simulink model "snap_sys_clk_feng"  (R2019a)
settings: Solver=VariableStepDiscrete  StartTime=0.0  StopTime=10.0  RelTol=1e-3
undefined symbols (not defined in the file): datetime, posixtime
libraries: xbsIndex_r4 x5252, casper_library_misc x69, xps_library x6, casper_library_delays x3
(part 13 of 45)

== system snap_sys_clk_feng/stats/calc_adc_sum_sq7 ==
  note: 127^2 == 16129
  in : Inport
  Accumulator : xbsIndex_r4/Accumulator  operation=Add  n_bits=32  overflow=Wrap  scale=1  rst=on  hasbypass=on  infoeditControl=reset for floating point data type must be asserted for a minimum of 2 cycles  en=off  latency=1  msb_inp=100  msb=100  lsb=-100  use_behavioral_HDL=on  implementation=Fabric  dbl_ovrd=off  block_type=accum
      settings: xl_area=[0, 0, 0, 0, 0, 0, 0]  block_version=10.1.3
  Accumulator1 : xbsIndex_r4/Accumulator  operation=Add  n_bits=32  overflow=Wrap  scale=1  rst=on  hasbypass=on  infoeditControl=reset for floating point data type must be asserted for a minimum of 2 cycles  en=off  latency=1  msb_inp=100  msb=100  lsb=-100  use_behavioral_HDL=on  implementation=Fabric  dbl_ovrd=off  block_type=accum
      settings: xl_area=[0, 0, 0, 0, 0, 0, 0]  block_version=10.1.3
  Accumulator2 : xbsIndex_r4/Accumulator  operation=Add  n_bits=32  overflow=Wrap  scale=1  rst=on  hasbypass=on  infoeditControl=reset for floating point data type must be asserted for a minimum of 2 cycles  en=off  latency=1  msb_inp=100  msb=100  lsb=-100  use_behavioral_HDL=on  implementation=Fabric  dbl_ovrd=off  block_type=accum
      settings: xl_area=[0, 0, 0, 0, 0, 0, 0]  block_version=10.1.3
  BitBasher : xbsIndex_r4/BitBasher  bitexpr=sss={clip, s, ss}  display_expr=off  sr_1=sss  arith_type1="Signed  (2's comp)"  bin_pt1=0  sr_2=2  arith_type2=Unsigned  bin_pt2=0  sr_3=3  arith_type3=Unsigned  bin_pt3=0  sr_4=4  arith_type4=Unsigned  bin_pt4=0  dbl_ovrd=off  block_type=bitbasher
      settings: block_version=10.1.3
  Constant : xbsIndex_r4/Constant  const=127^2  gui_display_data_type=Fixed-point  arith_type=Unsigned  n_bits=15  bin_pt=0  preci_type=Single  exp_width=8  frac_width=24  explicit_period=on  period=1  equ=P=C  opselect=C  inp2=PCIN>>17  opr=+  inp1=P  carry=CIN  dbl_ovrd=off  block_type=constant
  Delay : xbsIndex_r4/Delay  rst=off  infoeditControl=Selection of Reset will increase slice count due to use of real FFs and instead of SRLs  en=off  latency=2  reg_retiming=off  dbl_ovrd=off  block_type=delay
  Delay1 : xbsIndex_r4/Delay  rst=off  infoeditControl=Selection of Reset will increase slice count due to use of real FFs and instead of SRLs  en=off  latency=1  reg_retiming=off  dbl_ovrd=off  block_type=delay
  Delay2 : xbsIndex_r4/Delay  rst=off  infoeditControl=Selection of Reset will increase slice count due to use of real FFs and instead of SRLs  en=off  latency=1  reg_retiming=off  dbl_ovrd=off  block_type=delay
      settings: infoedit=Hardware notes: A delay line is a chain, each link of which is an SRL16 or SRL32 followed by a flip-flop.
  Mult : xbsIndex_r4/Mult  precision=User Defined  arith_type=Unsigned  n_bits=15  bin_pt=0  quantization=Truncate  overflow=Wrap  en=off  latency=2  use_behavioral_HDL=on  opt=Speed  use_embedded=on  optimum_pipeline=on  pipeline=on  dbl_ovrd=off  use_rpm=on  placement_style=Rectangular shape  block_type=mult
      settings: xl_area=[0, 0, 0, 0, 0, 0, 0]  block_version=10.1.3
  Register : xbsIndex_r4/Register  init=0  rst=off  en=on  dbl_ovrd=off  block_type=register
      settings: xl_area=[0, 0, 0, 0, 0, 0, 0]
  Register1 : xbsIndex_r4/Register  init=0  rst=off  en=on  dbl_ovrd=off  block_type=register
      settings: xl_area=[0, 0, 0, 0, 0, 0, 0]
  Register2 : xbsIndex_r4/Register  init=0  rst=off  en=on  dbl_ovrd=off  block_type=register
      settings: xl_area=[0, 0, 0, 0, 0, 0, 0]
  Reinterpret : xbsIndex_r4/Reinterpret  force_arith_type=off  arith_type=Unsigned  force_bin_pt=on  bin_pt=0  block_type=reinterpret
  Relational : xbsIndex_r4/Relational  mode=a>=b  op_type=Ufix  en=off  latency=0  dbl_ovrd=off  block_type=relational
  sum_sumsq : Outport
  wires:
  Register2/1 -> BitBasher/1
  Register/1 -> BitBasher/3
  Register1/1 -> BitBasher/2
  Accumulator2/1 -> Register2/1
  Delay2/1 -> Register/2, Register1/2, Register2/2, Accumulator/2, Accumulator1/2, Accumulator2/2
  Relational/1 -> Accumulator2/1
  Constant/1 -> Relational/2
  Reinterpret/1 -> Delay1/1
  Delay1/1 -> Delay/1, Mult/1, Mult/2
  BitBasher/1 -> sum_sumsq/1
  Delay/1 -> Accumulator1/1
  Accumulator1/1 -> Register1/1
  Mult/1 -> Relational/1, Accumulator/1
  Accumulator/1 -> Register/1
  [adc_rms_rst] -> Delay2/1
  in/1 -> Reinterpret/1

== system snap_sys_clk_feng/stats/calc_adc_sum_sq8 ==
  note: 127^2 == 16129
  in : Inport
  Accumulator : xbsIndex_r4/Accumulator  operation=Add  n_bits=32  overflow=Wrap  scale=1  rst=on  hasbypass=on  infoeditControl=reset for floating point data type must be asserted for a minimum of 2 cycles  en=off  latency=1  msb_inp=100  msb=100  lsb=-100  use_behavioral_HDL=on  implementation=Fabric  dbl_ovrd=off  block_type=accum
      settings: xl_area=[0, 0, 0, 0, 0, 0, 0]  block_version=10.1.3
  Accumulator1 : xbsIndex_r4/Accumulator  operation=Add  n_bits=32  overflow=Wrap  scale=1  rst=on  hasbypass=on  infoeditControl=reset for floating point data type must be asserted for a minimum of 2 cycles  en=off  latency=1  msb_inp=100  msb=100  lsb=-100  use_behavioral_HDL=on  implementation=Fabric  dbl_ovrd=off  block_type=accum
      settings: xl_area=[0, 0, 0, 0, 0, 0, 0]  block_version=10.1.3
  Accumulator2 : xbsIndex_r4/Accumulator  operation=Add  n_bits=32  overflow=Wrap  scale=1  rst=on  hasbypass=on  infoeditControl=reset for floating point data type must be asserted for a minimum of 2 cycles  en=off  latency=1  msb_inp=100  msb=100  lsb=-100  use_behavioral_HDL=on  implementation=Fabric  dbl_ovrd=off  block_type=accum
      settings: xl_area=[0, 0, 0, 0, 0, 0, 0]  block_version=10.1.3
  BitBasher : xbsIndex_r4/BitBasher  bitexpr=sss={clip, s, ss}  display_expr=off  sr_1=sss  arith_type1="Signed  (2's comp)"  bin_pt1=0  sr_2=2  arith_type2=Unsigned  bin_pt2=0  sr_3=3  arith_type3=Unsigned  bin_pt3=0  sr_4=4  arith_type4=Unsigned  bin_pt4=0  dbl_ovrd=off  block_type=bitbasher
      settings: block_version=10.1.3
  Constant : xbsIndex_r4/Constant  const=127^2  gui_display_data_type=Fixed-point  arith_type=Unsigned  n_bits=15  bin_pt=0  preci_type=Single  exp_width=8  frac_width=24  explicit_period=on  period=1  equ=P=C  opselect=C  inp2=PCIN>>17  opr=+  inp1=P  carry=CIN  dbl_ovrd=off  block_type=constant
  Delay : xbsIndex_r4/Delay  rst=off  infoeditControl=Selection of Reset will increase slice count due to use of real FFs and instead of SRLs  en=off  latency=2  reg_retiming=off  dbl_ovrd=off  block_type=delay
  Delay1 : xbsIndex_r4/Delay  rst=off  infoeditControl=Selection of Reset will increase slice count due to use of real FFs and instead of SRLs  en=off  latency=1  reg_retiming=off  dbl_ovrd=off  block_type=delay
  Delay2 : xbsIndex_r4/Delay  rst=off  infoeditControl=Selection of Reset will increase slice count due to use of real FFs and instead of SRLs  en=off  latency=1  reg_retiming=off  dbl_ovrd=off  block_type=delay
      settings: infoedit=Hardware notes: A delay line is a chain, each link of which is an SRL16 or SRL32 followed by a flip-flop.
  Mult : xbsIndex_r4/Mult  precision=User Defined  arith_type=Unsigned  n_bits=15  bin_pt=0  quantization=Truncate  overflow=Wrap  en=off  latency=2  use_behavioral_HDL=on  opt=Speed  use_embedded=on  optimum_pipeline=on  pipeline=on  dbl_ovrd=off  use_rpm=on  placement_style=Rectangular shape  block_type=mult
      settings: xl_area=[0, 0, 0, 0, 0, 0, 0]  block_version=10.1.3
  Register : xbsIndex_r4/Register  init=0  rst=off  en=on  dbl_ovrd=off  block_type=register
      settings: xl_area=[0, 0, 0, 0, 0, 0, 0]
  Register1 : xbsIndex_r4/Register  init=0  rst=off  en=on  dbl_ovrd=off  block_type=register
      settings: xl_area=[0, 0, 0, 0, 0, 0, 0]
  Register2 : xbsIndex_r4/Register  init=0  rst=off  en=on  dbl_ovrd=off  block_type=register
      settings: xl_area=[0, 0, 0, 0, 0, 0, 0]
  Reinterpret : xbsIndex_r4/Reinterpret  force_arith_type=off  arith_type=Unsigned  force_bin_pt=on  bin_pt=0  block_type=reinterpret
  Relational : xbsIndex_r4/Relational  mode=a>=b  op_type=Ufix  en=off  latency=0  dbl_ovrd=off  block_type=relational
  sum_sumsq : Outport
  wires:
  Register2/1 -> BitBasher/1
  Register/1 -> BitBasher/3
  Register1/1 -> BitBasher/2
  Accumulator2/1 -> Register2/1
  Delay2/1 -> Register/2, Register1/2, Register2/2, Accumulator/2, Accumulator1/2, Accumulator2/2
  Relational/1 -> Accumulator2/1
  Constant/1 -> Relational/2
  Reinterpret/1 -> Delay1/1
  Delay1/1 -> Delay/1, Mult/1, Mult/2
  BitBasher/1 -> sum_sumsq/1
  Delay/1 -> Accumulator1/1
  Accumulator1/1 -> Register1/1
  Mult/1 -> Relational/1, Accumulator/1
  Accumulator/1 -> Register/1
  [adc_rms_rst] -> Delay2/1
  in/1 -> Reinterpret/1

== system snap_sys_clk_feng/stats/calc_adc_sum_sq9 ==
  note: 127^2 == 16129
  in : Inport
  Accumulator : xbsIndex_r4/Accumulator  operation=Add  n_bits=32  overflow=Wrap  scale=1  rst=on  hasbypass=on  infoeditControl=reset for floating point data type must be asserted for a minimum of 2 cycles  en=off  latency=1  msb_inp=100  msb=100  lsb=-100  use_behavioral_HDL=on  implementation=Fabric  dbl_ovrd=off  block_type=accum
      settings: xl_area=[0, 0, 0, 0, 0, 0, 0]  block_version=10.1.3
  Accumulator1 : xbsIndex_r4/Accumulator  operation=Add  n_bits=32  overflow=Wrap  scale=1  rst=on  hasbypass=on  infoeditControl=reset for floating point data type must be asserted for a minimum of 2 cycles  en=off  latency=1  msb_inp=100  msb=100  lsb=-100  use_behavioral_HDL=on  implementation=Fabric  dbl_ovrd=off  block_type=accum
      settings: xl_area=[0, 0, 0, 0, 0, 0, 0]  block_version=10.1.3
  Accumulator2 : xbsIndex_r4/Accumulator  operation=Add  n_bits=32  overflow=Wrap  scale=1  rst=on  hasbypass=on  infoeditControl=reset for floating point data type must be asserted for a minimum of 2 cycles  en=off  latency=1  msb_inp=100  msb=100  lsb=-100  use_behavioral_HDL=on  implementation=Fabric  dbl_ovrd=off  block_type=accum
      settings: xl_area=[0, 0, 0, 0, 0, 0, 0]  block_version=10.1.3
  BitBasher : xbsIndex_r4/BitBasher  bitexpr=sss={clip, s, ss}  display_expr=off  sr_1=sss  arith_type1="Signed  (2's comp)"  bin_pt1=0  sr_2=2  arith_type2=Unsigned  bin_pt2=0  sr_3=3  arith_type3=Unsigned  bin_pt3=0  sr_4=4  arith_type4=Unsigned  bin_pt4=0  dbl_ovrd=off  block_type=bitbasher
      settings: block_version=10.1.3
  Constant : xbsIndex_r4/Constant  const=127^2  gui_display_data_type=Fixed-point  arith_type=Unsigned  n_bits=15  bin_pt=0  preci_type=Single  exp_width=8  frac_width=24  explicit_period=on  period=1  equ=P=C  opselect=C  inp2=PCIN>>17  opr=+  inp1=P  carry=CIN  dbl_ovrd=off  block_type=constant
  Delay : xbsIndex_r4/Delay  rst=off  infoeditControl=Selection of Reset will increase slice count due to use of real FFs and instead of SRLs  en=off  latency=2  reg_retiming=off  dbl_ovrd=off  block_type=delay
  Delay1 : xbsIndex_r4/Delay  rst=off  infoeditControl=Selection of Reset will increase slice count due to use of real FFs and instead of SRLs  en=off  latency=1  reg_retiming=off  dbl_ovrd=off  block_type=delay
  Delay2 : xbsIndex_r4/Delay  rst=off  infoeditControl=Selection of Reset will increase slice count due to use of real FFs and instead of SRLs  en=off  latency=1  reg_retiming=off  dbl_ovrd=off  block_type=delay
      settings: infoedit=Hardware notes: A delay line is a chain, each link of which is an SRL16 or SRL32 followed by a flip-flop.
  Mult : xbsIndex_r4/Mult  precision=User Defined  arith_type=Unsigned  n_bits=15  bin_pt=0  quantization=Truncate  overflow=Wrap  en=off  latency=2  use_behavioral_HDL=on  opt=Speed  use_embedded=on  optimum_pipeline=on  pipeline=on  dbl_ovrd=off  use_rpm=on  placement_style=Rectangular shape  block_type=mult
      settings: xl_area=[0, 0, 0, 0, 0, 0, 0]  block_version=10.1.3
  Register : xbsIndex_r4/Register  init=0  rst=off  en=on  dbl_ovrd=off  block_type=register
      settings: xl_area=[0, 0, 0, 0, 0, 0, 0]
  Register1 : xbsIndex_r4/Register  init=0  rst=off  en=on  dbl_ovrd=off  block_type=register
      settings: xl_area=[0, 0, 0, 0, 0, 0, 0]
  Register2 : xbsIndex_r4/Register  init=0  rst=off  en=on  dbl_ovrd=off  block_type=register
      settings: xl_area=[0, 0, 0, 0, 0, 0, 0]
  Reinterpret : xbsIndex_r4/Reinterpret  force_arith_type=off  arith_type=Unsigned  force_bin_pt=on  bin_pt=0  block_type=reinterpret
  Relational : xbsIndex_r4/Relational  mode=a>=b  op_type=Ufix  en=off  latency=0  dbl_ovrd=off  block_type=relational
  sum_sumsq : Outport
  wires:
  in/1 -> Reinterpret/1
  [adc_rms_rst] -> Delay2/1
  Accumulator/1 -> Register/1
  Mult/1 -> Accumulator/1, Relational/1
  Accumulator1/1 -> Register1/1
  Delay/1 -> Accumulator1/1
  BitBasher/1 -> sum_sumsq/1
  Delay1/1 -> Mult/2, Mult/1, Delay/1
  Reinterpret/1 -> Delay1/1
  Constant/1 -> Relational/2
  Relational/1 -> Accumulator2/1
  Delay2/1 -> Accumulator2/2, Accumulator1/2, Accumulator/2, Register2/2, Register1/2, Register/2
  Accumulator2/1 -> Register2/1
  Register1/1 -> BitBasher/2
  Register/1 -> BitBasher/3
  Register2/1 -> BitBasher/1

== system snap_sys_clk_feng/stats/edge_detect ==
  in : Inport
  Delay : xbsIndex_r4/Delay  rst=off  infoeditControl=Selection of Reset will increase slice count due to use of real FFs and instead of SRLs  en=off  latency=1  reg_retiming=off  dbl_ovrd=off  block_type=delay
      settings: xl_area=[0, 0, 0, 0, 0, 0, 0]
  Inverter : xbsIndex_r4/Inverter  en=off  latency=0  dbl_ovrd=off  block_type=inv
      settings: xl_area=[0, 0, 0, 0, 0, 0, 0]
  edge_op : xbsIndex_r4/Logical  logical_function=NOR  inputs=2  en=off  latency=0  precision=Full  arith_type=Unsigned  n_bits=8  bin_pt=2  align_bp=on  dbl_ovrd=off  block_type=logical
      settings: xl_area=[0, 0, 0, 0, 0, 0, 0]
  out : Outport
  wires:
  Inverter/1 -> edge_op/1
  edge_op/1 -> out/1
  in/1 -> Inverter/1, Delay/1
  Delay/1 -> edge_op/2

== system snap_sys_clk_feng/stats/enable ==
  sim_1 : Inport
  convert1_1 : DataTypeConversion  OutDataTypeStr=fixdt('ufix32_En0')  LockScale=on
  convert2_1 : DataTypeConversion  OutDataTypeStr=fixdt('ufix32_En0')  ConvertRealWorld=Stored Integer (SI)  LockScale=on
  gain_1 : Gain
  io_delay : xbsIndex_r4/Delay  rst=off  infoeditControl=Selection of Reset will increase slice count due to use of real FFs and instead of SRLs  en=off  latency=0  reg_retiming=on  dbl_ovrd=off  block_type=delay
  reint1 : xbsIndex_r4/Reinterpret  force_arith_type=on  arith_type=Unsigned  force_bin_pt=on  bin_pt=0  block_type=reinterpret
  slice_reg : xbsIndex_r4/Slice  nbits=32  boolean_output=off  mode=Lower Bit Location + Width  bit1=0  base1=MSB of Input  bit0=0  base0=LSB of Input  dbl_ovrd=off  block_type=slice
  snap_sys_clk_feng_stats_enable_user_data_out : xbsIndex_r4/Gateway In  gui_display_data_type=Fixed-point  arith_type=Unsigned  n_bits=32  bin_pt=0  preci_type=Single  exp_width=8  frac_width=24  rows=1  columns=1  quantization="Round  (unbiased: +/- Inf)"  overflow=Saturate  period=1  UseAsADC=off  ADCChannel='1'  interface=None  automatic_assignment=on  address_offset=hex2dec('00')  intf_name=''  intf_description=''  default_value=0  timing_constraint=None  locs_specified=off  LOCs={}  io_standard={}  inherit_from_input=off  hdl_port=on  dbl_ovrd=off  block_type=gatewayin
  in_reg : Outport
  wires:
  snap_sys_clk_feng_stats_enable_user_data_out/1 -> io_delay/1
  sim_1/1 -> convert1_1/1
  convert1_1/1 -> convert2_1/1
  convert2_1/1 -> gain_1/1
  gain_1/1 -> snap_sys_clk_feng_stats_enable_user_data_out/1
  io_delay/1 -> slice_reg/1
  slice_reg/1 -> reint1/1
  reint1/1 -> in_reg/1

== system snap_sys_clk_feng/stats/levels ==
  addr : Inport
  data_in : Inport  Port=2
  we : Inport  Port=3
  Terminator : Terminator
  Terminator1 : Terminator
  Terminator2 : Terminator
  calc_add : Subsystem  mask{data_width=128, addr_width=5, sample_rate=sample_rate}
      mask prompts: data_width "data width"; addr_width "address width"; sample_rate "sample rate"
  convert_addr : xbsIndex_r4/Convert  gui_display_data_type=Fixed-point  arith_type=Unsigned  n_bits=addr_width  bin_pt=0  float_type=Single  exp_bits=8  fraction_bits=24  quantization=Truncate  overflow=Wrap  en=off  latency=0  pipeline=off  dbl_ovrd=off  block_type=convert
      settings: xl_area=[0, 0, 0, 0, 0, 0, 0]
  convert_din1 : xbsIndex_r4/Convert  gui_display_data_type=Fixed-point  arith_type=Unsigned  n_bits=128  bin_pt=0  float_type=Single  exp_bits=8  fraction_bits=24  quantization=Truncate  overflow=Wrap  en=off  latency=0  pipeline=off  dbl_ovrd=off  block_type=convert
      settings: xl_area=[0, 0, 0, 0, 0, 0, 0]
  convert_we : xbsIndex_r4/Convert  gui_display_data_type=Fixed-point  arith_type=Unsigned  n_bits=1  bin_pt=0  float_type=Single  exp_bits=8  fraction_bits=24  quantization=Truncate  overflow=Wrap  en=off  latency=0  pipeline=off  dbl_ovrd=off  block_type=convert
      settings: xl_area=[0, 0, 0, 0, 0, 0, 0]
  munge_in : Subsystem  AncestorBlock=casper_library_flow_control/munge  mask(munge){divisions=4, div_size=[32 32 32 32], order=[3  2  1  0], arith_type_out=Unsigned, bin_pt_out=0}
      mask prompts: divisions "Number of divisions"; div_size "Division size (bits)"; order "Division packing order"; arith_type_out "Output arithmetic type"; bin_pt_out "Output binary point"
      mask help: Splits an input bus into the specified number of divisions and then recombines them in the order specified (most significant division = 0,least = number divisions-1)
      mask init:
      | munge_init(gcb, ...
      |     'divisions', divisions, ...
      |     'div_size', div_size, ...
      |     'order', order, ...
      |     'arith_type_out', arith_type_out, ...
      |     'bin_pt_out', bin_pt_out);
      settings: AttributesFormatString=|
      | split:[32 32 32 32]
      | join:[3 2 1 0]
      | Unsigned [128,0]
      mask TypeOptions arith_type_out: Unsigned | Signed  (2's comp) | Floating-point
  munge_out : Subsystem  AncestorBlock=casper_library_flow_control/munge  mask(munge){divisions=4, div_size=[32 32 32 32], order=[3  2  1  0], arith_type_out=Unsigned, bin_pt_out=0}
      mask prompts: divisions "Number of divisions"; div_size "Division size (bits)"; order "Division packing order"; arith_type_out "Output arithmetic type"; bin_pt_out "Output binary point"
      mask help: Splits an input bus into the specified number of divisions and then recombines them in the order specified (most significant division = 0,least = number divisions-1)
      mask init:
      | munge_init(gcb, ...
      |     'divisions', divisions, ...
      |     'div_size', div_size, ...
      |     'order', order, ...
      |     'arith_type_out', arith_type_out, ...
      |     'bin_pt_out', bin_pt_out);
      settings: AttributesFormatString=|
      | split:[32 32 32 32]
      | join:[3 2 1 0]
      | Unsigned [128,0]
      mask TypeOptions arith_type_out: Unsigned | Signed  (2's comp) | Floating-point
  sim_mem : Subsystem  mask{arith_type=Unsigned, addr_width=5, data_width=128, data_bin_pt=0, init_vals=[0   1   2   3   4   5   6   7   8   9  10  11  12  13  14  15  16  17  18  19  20  21  22  23  24  25  26  27  28  29  30  31], sample_rate=1, csp_latency=3}
      mask prompts: arith_type "Output Data Type"; addr_width "Address width"; data_width "Data width"; data_bin_pt "Data Binary Point"; init_vals "Initial values"; sample_rate "Sample rate"; csp_latency "Latency"
      mask init:
      | % set_param([gcb, '/data_to_xilinx'], 'arith_type', arith_type)
      | % set_param([gcb, '/data_to_xilinx'], 'n_bits', get_param(gcb, 'data_width'))
      mask TypeOptions arith_type: Unsigned | Signed  (2's comp)
      mask TypeOptions data_width: 8 | 16 | 32 | 64 | 128
  snap_sys_clk_feng_stats_levels_addr : xbsIndex_r4/Gateway Out  inherit_from_input=off  hdl_port=on  rows=1  columns=1  UseAsDAC=off  DACChannel='1'  interface=None  automatic_assignment=on  address_offset=hex2dec('00')  intf_name=''  intf_description=''  timing_constraint=None  locs_specified=off  LOCs={'A5','B9','A9','C1','A3','G6','E9','A6','A7','A8','B8','B1','B3','D9','B5','B4','B6','C2'}  io_standard={}  block_type=gatewayout
      settings: infoedit="Gateway out block.  Converts Xilinx fixed point inputs into ouputs of type Simulink integer, double, or fixed point.<P><P>Hardware notes:  In hardware these blocks become top level output ports or are discarded, depending on how they are configured."  sginterface={'Nallatech'=>{'xdspkit'=>{'non_memory_mapped_port'=>'uprev_Shared_BRAM_addr'}},'Xilinx'=>{'jtaghwcosim'=>{'non_memory_mapped_port'=>'uprev_Shared_BRAM_addr'},'xdspkit'=>{'non_memory_mapped_port'=>'uprev_Shared_BRAM_addr'}}}  xl_area=[0, 0, 0, 0, 0, 0, 0]
  snap_sys_clk_feng_stats_levels_data_in : xbsIndex_r4/Gateway Out  inherit_from_input=off  hdl_port=on  rows=1  columns=1  UseAsDAC=off  DACChannel='1'  interface=None  automatic_assignment=on  address_offset=hex2dec('00')  intf_name=''  intf_description=''  timing_constraint=None  locs_specified=off  LOCs={'B21','B22','A22','B23','B19','C19','A20','A21','A23','B24','A24','A25','E18','D18','C18','B18'}  io_standard={}  block_type=gatewayout
      settings: infoedit="Gateway out block.  Converts Xilinx fixed point inputs into ouputs of type Simulink integer, double, or fixed point.<P><P>Hardware notes:  In hardware these blocks become top level output ports or are discarded, depending on how they are configured."  sginterface={'Nallatech'=>{'xdspkit'=>{'non_memory_mapped_port'=>'uprev_Shared_BRAM_data_in'}},'Xilinx'=>{'jtaghwcosim'=>{'non_memory_mapped_port'=>'uprev_Shared_BRAM_data_in'},'xdspkit'=>{'non_memory_mapped_port'=>'uprev_Shared_BRAM_data_in'}}}  xl_area=[0, 0, 0, 0, 0, 0, 0]
  snap_sys_clk_feng_stats_levels_data_out : xbsIndex_r4/Gateway In  gui_display_data_type=Fixed-point  arith_type=Unsigned  n_bits=128  bin_pt=0  preci_type=Single  exp_width=8  frac_width=24  rows=1  columns=1  quantization=Truncate  overflow=Wrap  period=sample_rate  UseAsADC=off  ADCChannel='1'  interface=None  automatic_assignment=on  address_offset=hex2dec('00')  intf_name=''  intf_description=''  default_value=0  timing_constraint=None  locs_specified=off  LOCs={}  io_standard={}  inherit_from_input=off  hdl_port=on  dbl_ovrd=off  block_type=gatewayin
      settings: xl_area=[0, 0, 0, 0, 0, 0, 0]
  snap_sys_clk_feng_stats_levels_we : xbsIndex_r4/Gateway Out  inherit_from_input=off  hdl_port=on  rows=1  columns=1  UseAsDAC=off  DACChannel='1'  interface=None  automatic_assignment=on  address_offset=hex2dec('00')  intf_name=''  intf_description=''  timing_constraint=None  locs_specified=off  LOCs={'A14'}  io_standard={}  block_type=gatewayout
      settings: infoedit="Gateway out block.  Converts Xilinx fixed point inputs into ouputs of type Simulink integer, double, or fixed point.<P><P>Hardware notes:  In hardware these blocks become top level output ports or are discarded, depending on how they are configured."  xl_area=[0, 0, 0, 0, 0, 0, 0]
  data_out : Outport
  wires:
  munge_out/1(dout) -> data_out/1
  sim_mem/1(data_out) -> snap_sys_clk_feng_stats_levels_data_out/1
  snap_sys_clk_feng_stats_levels_data_out/1 -> munge_out/1(din)
  convert_addr/1 -> snap_sys_clk_feng_stats_levels_addr/1
  convert_din1/1 -> snap_sys_clk_feng_stats_levels_data_in/1
  data_in/1 -> munge_in/1(din)
  calc_add/1(out) -> sim_mem/1(addr), convert_addr/1
  snap_sys_clk_feng_stats_levels_we/1 -> Terminator2/1
  snap_sys_clk_feng_stats_levels_data_in/1 -> Terminator1/1
  snap_sys_clk_feng_stats_levels_addr/1 -> Terminator/1
  convert_we/1 -> snap_sys_clk_feng_stats_levels_we/1
  addr/1 -> calc_add/1(in)
  we/1 -> sim_mem/3(we), convert_we/1
  munge_in/1(dout) -> sim_mem/2(data), convert_din1/1

== system snap_sys_clk_feng/sync/arm ==
  sim_1 : Inport
  convert1_1 : DataTypeConversion  OutDataTypeStr=fixdt('ufix32_En0')  LockScale=on
  convert2_1 : DataTypeConversion  OutDataTypeStr=fixdt('ufix32_En0')  ConvertRealWorld=Stored Integer (SI)  LockScale=on
  gain_1 : Gain
  io_delay : xbsIndex_r4/Delay  rst=off  infoeditControl=Selection of Reset will increase slice count due to use of real FFs and instead of SRLs  en=off  latency=0  reg_retiming=on  dbl_ovrd=off  block_type=delay
  reint1 : xbsIndex_r4/Reinterpret  force_arith_type=on  arith_type=Unsigned  force_bin_pt=on  bin_pt=0  block_type=reinterpret
  slice_reg : xbsIndex_r4/Slice  nbits=32  boolean_output=off  mode=Lower Bit Location + Width  bit1=0  base1=MSB of Input  bit0=0  base0=LSB of Input  dbl_ovrd=off  block_type=slice
  snap_sys_clk_feng_sync_arm_user_data_out : xbsIndex_r4/Gateway In  gui_display_data_type=Fixed-point  arith_type=Unsigned  n_bits=32  bin_pt=0  preci_type=Single  exp_width=8  frac_width=24  rows=1  columns=1  quantization="Round  (unbiased: +/- Inf)"  overflow=Saturate  period=1  UseAsADC=off  ADCChannel='1'  interface=None  automatic_assignment=on  address_offset=hex2dec('00')  intf_name=''  intf_description=''  default_value=0  timing_constraint=None  locs_specified=off  LOCs={}  io_standard={}  inherit_from_input=off  hdl_port=on  dbl_ovrd=off  block_type=gatewayin
  in_reg : Outport
  wires:
  snap_sys_clk_feng_sync_arm_user_data_out/1 -> io_delay/1
  sim_1/1 -> convert1_1/1
  convert1_1/1 -> convert2_1/1
  convert2_1/1 -> gain_1/1
  gain_1/1 -> snap_sys_clk_feng_sync_arm_user_data_out/1
  io_delay/1 -> slice_reg/1
  slice_reg/1 -> reint1/1
  reint1/1 -> in_reg/1

== system snap_sys_clk_feng/sync/count ==
  out_reg : Inport
  assert_reg : xbsIndex_r4/Assert  assert_type=on  type_source=Explicitly  gui_display_data_type=Fixed-point  arith_type=Unsigned  n_bits=32  bin_pt=0  preci_type=Single  exp_width=8  frac_width=24  assert_rate=off  rate_source=Explicitly  period=1  output_port=on  block_type=assert
  cast_gw : xbsIndex_r4/Convert  gui_display_data_type=Fixed-point  arith_type=Unsigned  n_bits=32  bin_pt=0  float_type=Single  exp_bits=8  fraction_bits=24  quantization=Truncate  overflow=Wrap  en=off  latency=1  pipeline=off  dbl_ovrd=off  block_type=convert
  io_delay : xbsIndex_r4/Delay  rst=off  infoeditControl=Selection of Reset will increase slice count due to use of real FFs and instead of SRLs  en=off  latency=0  reg_retiming=on  dbl_ovrd=off  block_type=delay
  reint1 : xbsIndex_r4/Reinterpret  force_arith_type=on  arith_type=Unsigned  force_bin_pt=on  bin_pt=0  block_type=reinterpret
  sim_out : Terminator
  sim_out_reg_gw : xbsIndex_r4/Gateway Out  inherit_from_input=off  hdl_port=off  rows=1  columns=1  UseAsDAC=off  DACChannel='1'  interface=None  automatic_assignment=on  address_offset=hex2dec('00')  intf_name=''  intf_description=''  timing_constraint=None  locs_specified=off  LOCs={}  io_standard={}  block_type=gatewayout
  sim_out_reg_sim_delay : xbsIndex_r4/Delay  rst=off  infoeditControl=Selection of Reset will increase slice count due to use of real FFs and instead of SRLs  en=off  latency=1  reg_retiming=on  dbl_ovrd=off  block_type=delay
  snap_sys_clk_feng_sync_count_user_data_in : xbsIndex_r4/Gateway Out  inherit_from_input=off  hdl_port=on  rows=1  columns=1  UseAsDAC=off  DACChannel='1'  interface=None  automatic_assignment=on  address_offset=hex2dec('00')  intf_name=''  intf_description=''  timing_constraint=None  locs_specified=off  LOCs={}  io_standard={}  block_type=gatewayout
  sim_out_reg : Outport
  wires:
  sim_out_reg_sim_delay/1 -> sim_out_reg_gw/1
  sim_out_reg_gw/1 -> sim_out_reg/1
  io_delay/1 -> cast_gw/1
  cast_gw/1 -> snap_sys_clk_feng_sync_count_user_data_in/1
  snap_sys_clk_feng_sync_count_user_data_in/1 -> sim_out/1
  out_reg/1 -> sim_out_reg_sim_delay/1, assert_reg/1
  assert_reg/1 -> reint1/1
  reint1/1 -> io_delay/1

== system snap_sys_clk_feng/sync/edge_detect ==
  in : Inport
  Delay : xbsIndex_r4/Delay  rst=off  infoeditControl=Selection of Reset will increase slice count due to use of real FFs and instead of SRLs  en=off  latency=1  reg_retiming=off  dbl_ovrd=off  block_type=delay
      settings: xl_area=[0, 0, 0, 0, 0, 0, 0]
  Inverter : xbsIndex_r4/Inverter  en=off  latency=0  dbl_ovrd=off  block_type=inv
      settings: xl_area=[0, 0, 0, 0, 0, 0, 0]
  edge_op : xbsIndex_r4/Logical  logical_function=NOR  inputs=2  en=off  latency=0  precision=Full  arith_type=Unsigned  n_bits=8  bin_pt=2  align_bp=on  dbl_ovrd=off  block_type=logical
      settings: xl_area=[0, 0, 0, 0, 0, 0, 0]
  out : Outport
  wires:
  Inverter/1 -> edge_op/1
  edge_op/1 -> out/1
  in/1 -> Inverter/1, Delay/1
  Delay/1 -> edge_op/2

== system snap_sys_clk_feng/sync/edge_detect1 ==
  in : Inport
  Delay : xbsIndex_r4/Delay  rst=off  infoeditControl=Selection of Reset will increase slice count due to use of real FFs and instead of SRLs  en=off  latency=1  reg_retiming=off  dbl_ovrd=off  block_type=delay
      settings: xl_area=[0, 0, 0, 0, 0, 0, 0]
  Inverter : xbsIndex_r4/Inverter  en=off  latency=0  dbl_ovrd=off  block_type=inv
      settings: xl_area=[0, 0, 0, 0, 0, 0, 0]
  edge_op : xbsIndex_r4/Logical  logical_function=AND  inputs=2  en=off  latency=0  precision=Full  arith_type=Unsigned  n_bits=8  bin_pt=2  align_bp=on  dbl_ovrd=off  block_type=logical
      settings: xl_area=[0, 0, 0, 0, 0, 0, 0]
  out : Outport
  wires:
  Inverter/1 -> edge_op/1
  edge_op/1 -> out/1
  in/1 -> Inverter/1, Delay/1
  Delay/1 -> edge_op/2

== system snap_sys_clk_feng/sync/edge_detect2 ==
  in : Inport
  Delay : xbsIndex_r4/Delay  rst=off  infoeditControl=Selection of Reset will increase slice count due to use of real FFs and instead of SRLs  en=off  latency=1  reg_retiming=off  dbl_ovrd=off  block_type=delay
      settings: xl_area=[0, 0, 0, 0, 0, 0, 0]
  Inverter : xbsIndex_r4/Inverter  en=off  latency=0  dbl_ovrd=off  block_type=inv
      settings: xl_area=[0, 0, 0, 0, 0, 0, 0]
  edge_op : xbsIndex_r4/Logical  logical_function=NOR  inputs=2  en=off  latency=0  precision=Full  arith_type=Unsigned  n_bits=8  bin_pt=2  align_bp=on  dbl_ovrd=off  block_type=logical
      settings: xl_area=[0, 0, 0, 0, 0, 0, 0]
  out : Outport
  wires:
  Delay/1 -> edge_op/2
  in/1 -> Delay/1, Inverter/1
  edge_op/1 -> out/1
  Inverter/1 -> edge_op/1

== system snap_sys_clk_feng/sync/edge_detect3 ==
  in : Inport
  Delay : xbsIndex_r4/Delay  rst=off  infoeditControl=Selection of Reset will increase slice count due to use of real FFs and instead of SRLs  en=off  latency=1  reg_retiming=off  dbl_ovrd=off  block_type=delay
      settings: xl_area=[0, 0, 0, 0, 0, 0, 0]
  Inverter : xbsIndex_r4/Inverter  en=off  latency=0  dbl_ovrd=off  block_type=inv
      settings: xl_area=[0, 0, 0, 0, 0, 0, 0]
  edge_op : xbsIndex_r4/Logical  logical_function=NOR  inputs=2  en=off  latency=0  precision=Full  arith_type=Unsigned  n_bits=8  bin_pt=2  align_bp=on  dbl_ovrd=off  block_type=logical
      settings: xl_area=[0, 0, 0, 0, 0, 0, 0]
  out : Outport
  wires:
  Delay/1 -> edge_op/2
  in/1 -> Delay/1, Inverter/1
  edge_op/1 -> out/1
  Inverter/1 -> edge_op/1

== system snap_sys_clk_feng/sync/period ==
  out_reg : Inport
  assert_reg : xbsIndex_r4/Assert  assert_type=on  type_source=Explicitly  gui_display_data_type=Fixed-point  arith_type=Unsigned  n_bits=32  bin_pt=0  preci_type=Single  exp_width=8  frac_width=24  assert_rate=off  rate_source=Explicitly  period=1  output_port=on  block_type=assert
  cast_gw : xbsIndex_r4/Convert  gui_display_data_type=Fixed-point  arith_type=Unsigned  n_bits=32  bin_pt=0  float_type=Single  exp_bits=8  fraction_bits=24  quantization=Truncate  overflow=Wrap  en=off  latency=1  pipeline=off  dbl_ovrd=off  block_type=convert
  io_delay : xbsIndex_r4/Delay  rst=off  infoeditControl=Selection of Reset will increase slice count due to use of real FFs and instead of SRLs  en=off  latency=0  reg_retiming=on  dbl_ovrd=off  block_type=delay
  reint1 : xbsIndex_r4/Reinterpret  force_arith_type=on  arith_type=Unsigned  force_bin_pt=on  bin_pt=0  block_type=reinterpret
  sim_out : Terminator
  sim_out_reg_gw : xbsIndex_r4/Gateway Out  inherit_from_input=off  hdl_port=off  rows=1  columns=1  UseAsDAC=off  DACChannel='1'  interface=None  automatic_assignment=on  address_offset=hex2dec('00')  intf_name=''  intf_description=''  timing_constraint=None  locs_specified=off  LOCs={}  io_standard={}  block_type=gatewayout
  sim_out_reg_sim_delay : xbsIndex_r4/Delay  rst=off  infoeditControl=Selection of Reset will increase slice count due to use of real FFs and instead of SRLs  en=off  latency=1  reg_retiming=on  dbl_ovrd=off  block_type=delay
  snap_sys_clk_feng_sync_period_user_data_in : xbsIndex_r4/Gateway Out  inherit_from_input=off  hdl_port=on  rows=1  columns=1  UseAsDAC=off  DACChannel='1'  interface=None  automatic_assignment=on  address_offset=hex2dec('00')  intf_name=''  intf_description=''  timing_constraint=None  locs_specified=off  LOCs={}  io_standard={}  block_type=gatewayout
  sim_out_reg : Outport
  wires:
  sim_out_reg_sim_delay/1 -> sim_out_reg_gw/1
  sim_out_reg_gw/1 -> sim_out_reg/1
  io_delay/1 -> cast_gw/1
  cast_gw/1 -> snap_sys_clk_feng_sync_period_user_data_in/1
  snap_sys_clk_feng_sync_period_user_data_in/1 -> sim_out/1
  out_reg/1 -> sim_out_reg_sim_delay/1, assert_reg/1
  assert_reg/1 -> reint1/1
  reint1/1 -> io_delay/1

== system snap_sys_clk_feng/sync/sel ==
  sim_1 : Inport
  convert1_1 : DataTypeConversion  OutDataTypeStr=fixdt('ufix1_En0')  LockScale=on
  convert2_1 : DataTypeConversion  OutDataTypeStr=fixdt('ufix1_En0')  ConvertRealWorld=Stored Integer (SI)  LockScale=on
  gain_1 : Gain
  io_delay : xbsIndex_r4/Delay  rst=off  infoeditControl=Selection of Reset will increase slice count due to use of real FFs and instead of SRLs  en=off  latency=0  reg_retiming=on  dbl_ovrd=off  block_type=delay
  reint1 : xbsIndex_r4/Reinterpret  force_arith_type=on  arith_type=Unsigned  force_bin_pt=on  bin_pt=0  block_type=reinterpret
  slice_reg : xbsIndex_r4/Slice  nbits=1  boolean_output=off  mode=Lower Bit Location + Width  bit1=0  base1=MSB of Input  bit0=0  base0=LSB of Input  dbl_ovrd=off  block_type=slice
  snap_sys_clk_feng_sync_sel_user_data_out : xbsIndex_r4/Gateway In  gui_display_data_type=Fixed-point  arith_type=Unsigned  n_bits=32  bin_pt=0  preci_type=Single  exp_width=8  frac_width=24  rows=1  columns=1  quantization="Round  (unbiased: +/- Inf)"  overflow=Saturate  period=1  UseAsADC=off  ADCChannel='1'  interface=None  automatic_assignment=on  address_offset=hex2dec('00')  intf_name=''  intf_description=''  default_value=0  timing_constraint=None  locs_specified=off  LOCs={}  io_standard={}  inherit_from_input=off  hdl_port=on  dbl_ovrd=off  block_type=gatewayin
  in_reg : Outport
  wires:
  snap_sys_clk_feng_sync_sel_user_data_out/1 -> io_delay/1
  sim_1/1 -> convert1_1/1
  convert1_1/1 -> convert2_1/1
  convert2_1/1 -> gain_1/1
  gain_1/1 -> snap_sys_clk_feng_sync_sel_user_data_out/1
  io_delay/1 -> slice_reg/1
  slice_reg/1 -> reint1/1
  reint1/1 -> in_reg/1

== system snap_sys_clk_feng/sync/sync_time ==
  sim_1 : Inport
  convert1_1 : DataTypeConversion  OutDataTypeStr=fixdt('ufix32_En0')  LockScale=on
  convert2_1 : DataTypeConversion  OutDataTypeStr=fixdt('ufix32_En0')  ConvertRealWorld=Stored Integer (SI)  LockScale=on
  gain_1 : Gain
  io_delay : xbsIndex_r4/Delay  rst=off  infoeditControl=Selection of Reset will increase slice count due to use of real FFs and instead of SRLs  en=off  latency=0  reg_retiming=on  dbl_ovrd=off  block_type=delay
  reint1 : xbsIndex_r4/Reinterpret  force_arith_type=on  arith_type=Unsigned  force_bin_pt=on  bin_pt=0  block_type=reinterpret
  slice_reg : xbsIndex_r4/Slice  nbits=32  boolean_output=off  mode=Lower Bit Location + Width  bit1=0  base1=MSB of Input  bit0=0  base0=LSB of Input  dbl_ovrd=off  block_type=slice
  snap_sys_clk_feng_sync_sync_time_user_data_out : xbsIndex_r4/Gateway In  gui_display_data_type=Fixed-point  arith_type=Unsigned  n_bits=32  bin_pt=0  preci_type=Single  exp_width=8  frac_width=24  rows=1  columns=1  quantization="Round  (unbiased: +/- Inf)"  overflow=Saturate  period=1  UseAsADC=off  ADCChannel='1'  interface=None  automatic_assignment=on  address_offset=hex2dec('00')  intf_name=''  intf_description=''  default_value=0  timing_constraint=None  locs_specified=off  LOCs={}  io_standard={}  inherit_from_input=off  hdl_port=on  dbl_ovrd=off  block_type=gatewayin
  in_reg : Outport
  wires:
  snap_sys_clk_feng_sync_sync_time_user_data_out/1 -> io_delay/1
  sim_1/1 -> convert1_1/1
  convert1_1/1 -> convert2_1/1
  convert2_1/1 -> gain_1/1
  gain_1/1 -> snap_sys_clk_feng_sync_sync_time_user_data_out/1
  io_delay/1 -> slice_reg/1
  slice_reg/1 -> reint1/1
  reint1/1 -> in_reg/1

== system snap_sys_clk_feng/sync/uptime ==
  out_reg : Inport
  assert_reg : xbsIndex_r4/Assert  assert_type=on  type_source=Explicitly  gui_display_data_type=Fixed-point  arith_type=Unsigned  n_bits=32  bin_pt=0  preci_type=Single  exp_width=8  frac_width=24  assert_rate=off  rate_source=Explicitly  period=1  output_port=on  block_type=assert
  cast_gw : xbsIndex_r4/Convert  gui_display_data_type=Fixed-point  arith_type=Unsigned  n_bits=32  bin_pt=0  float_type=Single  exp_bits=8  fraction_bits=24  quantization=Truncate  overflow=Wrap  en=off  latency=1  pipeline=off  dbl_ovrd=off  block_type=convert
  io_delay : xbsIndex_r4/Delay  rst=off  infoeditControl=Selection of Reset will increase slice count due to use of real FFs and instead of SRLs  en=off  latency=0  reg_retiming=on  dbl_ovrd=off  block_type=delay
  reint1 : xbsIndex_r4/Reinterpret  force_arith_type=on  arith_type=Unsigned  force_bin_pt=on  bin_pt=0  block_type=reinterpret
  sim_out : Terminator
  sim_out_reg_gw : xbsIndex_r4/Gateway Out  inherit_from_input=off  hdl_port=off  rows=1  columns=1  UseAsDAC=off  DACChannel='1'  interface=None  automatic_assignment=on  address_offset=hex2dec('00')  intf_name=''  intf_description=''  timing_constraint=None  locs_specified=off  LOCs={}  io_standard={}  block_type=gatewayout
  sim_out_reg_sim_delay : xbsIndex_r4/Delay  rst=off  infoeditControl=Selection of Reset will increase slice count due to use of real FFs and instead of SRLs  en=off  latency=1  reg_retiming=on  dbl_ovrd=off  block_type=delay
  snap_sys_clk_feng_sync_uptime_user_data_in : xbsIndex_r4/Gateway Out  inherit_from_input=off  hdl_port=on  rows=1  columns=1  UseAsDAC=off  DACChannel='1'  interface=None  automatic_assignment=on  address_offset=hex2dec('00')  intf_name=''  intf_description=''  timing_constraint=None  locs_specified=off  LOCs={}  io_standard={}  block_type=gatewayout
  sim_out_reg : Outport
  wires:
  sim_out_reg_sim_delay/1 -> sim_out_reg_gw/1
  sim_out_reg_gw/1 -> sim_out_reg/1
  io_delay/1 -> cast_gw/1
  cast_gw/1 -> snap_sys_clk_feng_sync_uptime_user_data_in/1
  snap_sys_clk_feng_sync_uptime_user_data_in/1 -> sim_out/1
  out_reg/1 -> sim_out_reg_sim_delay/1, assert_reg/1
  assert_reg/1 -> reint1/1
  reint1/1 -> io_delay/1

== system snap_sys_clk_feng/timebase/sync_period ==
  sim_1 : Inport
  convert1_1 : DataTypeConversion  OutDataTypeStr=fixdt('ufix32_En0')  LockScale=on
  convert2_1 : DataTypeConversion  OutDataTypeStr=fixdt('ufix32_En0')  ConvertRealWorld=Stored Integer (SI)  LockScale=on
  gain_1 : Gain
  io_delay : xbsIndex_r4/Delay  rst=off  infoeditControl=Selection of Reset will increase slice count due to use of real FFs and instead of SRLs  en=off  latency=0  reg_retiming=on  dbl_ovrd=off  block_type=delay
  reint1 : xbsIndex_r4/Reinterpret  force_arith_type=on  arith_type=Unsigned  force_bin_pt=on  bin_pt=0  block_type=reinterpret
  slice_reg : xbsIndex_r4/Slice  nbits=32  boolean_output=off  mode=Lower Bit Location + Width  bit1=0  base1=MSB of Input  bit0=0  base0=LSB of Input  dbl_ovrd=off  block_type=slice
  snap_sys_clk_feng_timebase_sync_period_user_data_out : xbsIndex_r4/Gateway In  gui_display_data_type=Fixed-point  arith_type=Unsigned  n_bits=32  bin_pt=0  preci_type=Single  exp_width=8  frac_width=24  rows=1  columns=1  quantization="Round  (unbiased: +/- Inf)"  overflow=Saturate  period=1  UseAsADC=off  ADCChannel='1'  interface=None  automatic_assignment=on  address_offset=hex2dec('00')  intf_name=''  intf_description=''  default_value=0  timing_constraint=None  locs_specified=off  LOCs={}  io_standard={}  inherit_from_input=off  hdl_port=on  dbl_ovrd=off  block_type=gatewayin
  in_reg : Outport
  wires:
  snap_sys_clk_feng_timebase_sync_period_user_data_out/1 -> io_delay/1
  sim_1/1 -> convert1_1/1
  convert1_1/1 -> convert2_1/1
  convert2_1/1 -> gain_1/1
  gain_1/1 -> snap_sys_clk_feng_timebase_sync_period_user_data_out/1
  io_delay/1 -> slice_reg/1
  slice_reg/1 -> reint1/1
  reint1/1 -> in_reg/1

== system snap_sys_clk_feng/timebase/timing ==
  note: On arm rising edge
      | raises armed till specified
      | number of ppss seen.
  note: Generates sync one
      | clk cycle after rst
      | lowered. Syncs
      | produced with
      | specified period
  arm : Inport
  data_in : Inport  Port=2
  sync_period : Inport  Port=3
  pps_in : Inport  Port=4
  Delay : xbsIndex_r4/Delay  rst=off  infoeditControl=Selection of Reset will increase slice count due to use of real FFs and instead of SRLs  en=off  latency=1  reg_retiming=off  dbl_ovrd=off  block_type=delay
      settings: block_version=11.4
  Delay1 : xbsIndex_r4/Delay  rst=off  infoeditControl=Selection of Reset will increase slice count due to use of real FFs and instead of SRLs  en=off  latency=1  reg_retiming=off  dbl_ovrd=off  block_type=delay
      settings: block_version=11.4
  Delay2 : xbsIndex_r4/Delay  rst=off  infoeditControl=Selection of Reset will increase slice count due to use of real FFs and instead of SRLs  en=off  latency=1  reg_retiming=off  dbl_ovrd=off  block_type=delay
      settings: block_version=11.4
  Slice : xbsIndex_r4/Slice  nbits=sync_gen_bits  boolean_output=off  mode=Lower Bit Location + Width  bit1=0  base1=MSB of Input  bit0=0  base0=LSB of Input  dbl_ovrd=off  block_type=slice
      settings: infoedit="Extracts a given range of bits from each input sample and presents it at the output.  The output type is ordinarily unsigned with binary point at zero, but can be Boolean when the slice is one bit wide.<P><P>Hardware notes: In hardware this block costs nothing."  block_version=10.1.3
  rst_gen : Subsystem  mask{reset_period=reset_period}
      mask prompts: reset_period "Min period of reset (pps pulses)"
      mask init:
      | %reset_period = eval(get_param(gcb,'reset_period'))
      | %bits = ceil(log2(reset_period))
      | %set_param([gcb,'/Counter'],'n_bits',num2str(bits));
      | %set_param([gcb,'/Counter'],'start_count', num2str(reset_period))
      | %set_param([gcb,'/Constant'],'n_bits',num2str(bits));
  sync_gen : Subsystem  mask{sync_gen_bits=sync_gen_bits}
      mask prompts: sync_gen_bits "Size of sync generator counter"
  armed : Outport
  sync : Outport  Port=2
  data_out : Outport  Port=3
  wires:
  arm/1 -> rst_gen/1(arm)
  data_in/1 -> rst_gen/3(din)
  pps_in/1 -> rst_gen/2(pps_in)
  sync_period/1 -> Slice/1
  rst_gen/1(mrst) -> Delay2/1, sync_gen/1(rst)
  sync_gen/1(sync) -> Delay1/1
  Slice/1 -> sync_gen/2(sync_period)
  sync_gen/2(dout) -> Delay/1
  rst_gen/2(dout) -> sync_gen/3(din)
  Delay/1 -> data_out/1
  Delay1/1 -> sync/1
  Delay2/1 -> armed/1

== system snap_sys_clk_feng/chan_reorder/demux/bus_expand1 ==
  bus_in : Inport
  reinterpret1 : xbsIndex_r4/Reinterpret  force_arith_type=on  arith_type=Unsigned  force_bin_pt=on  bin_pt=0  block_type=reinterpret
  reinterpret2 : xbsIndex_r4/Reinterpret  force_arith_type=on  arith_type=Unsigned  force_bin_pt=on  bin_pt=0  block_type=reinterpret
  slice1 : xbsIndex_r4/Slice  nbits=64  boolean_output=off  mode=Upper Bit Location + Width  bit1=-64  base1=MSB of Input  bit0=0  base0=LSB of Input  dbl_ovrd=off  block_type=slice
  slice2 : xbsIndex_r4/Slice  nbits=64  boolean_output=off  mode=Upper Bit Location + Width  bit1=0  base1=MSB of Input  bit0=0  base0=LSB of Input  dbl_ovrd=off  block_type=slice
  msb_out2 : Outport
  lsb_out1 : Outport  Port=2
  wires:
  bus_in/1 -> slice2/1, slice1/1
  slice2/1 -> reinterpret2/1
  reinterpret2/1 -> msb_out2/1
  slice1/1 -> reinterpret1/1
  reinterpret1/1 -> lsb_out1/1
